simulink model "pvwindupfc11"  (R2016a)
settings: Solver=VariableStepAuto  StartTime=0.0  StopTime=0.5  RelTol=1e-3
undefined symbols (not defined in the file): BCMS11, c1, c2, c3, c4, c5, c6, Clink_3L, DiscIntNeverNeededParam, fdesignblkfcn, Fnom, gcbh, Ion, Ki_Ireg_3L, Ki_VDCreg_3L, Kp_Ireg_3L, Kp_VDCreg_3L, LimitL_Ireg_3L, LimitL_VDCreg_3L, LimitU_Ireg_3L, LimitU_VDCreg_3L, Lithium, LowerLimit, Pnom_3L, Pnom_dc_3L, PV11, Ts_Control, Ts_Power, Ts_PWM, UpperLimit, Vnom_dc_3L, Vnom_prim_3L, Vnom_sec_3L
libraries: powerlib x98, powerlib_extras x29, powerlib_meascontrol x20, fuzblock x2, simulink x1, electricdrivelib x1
(part 3 of 4)

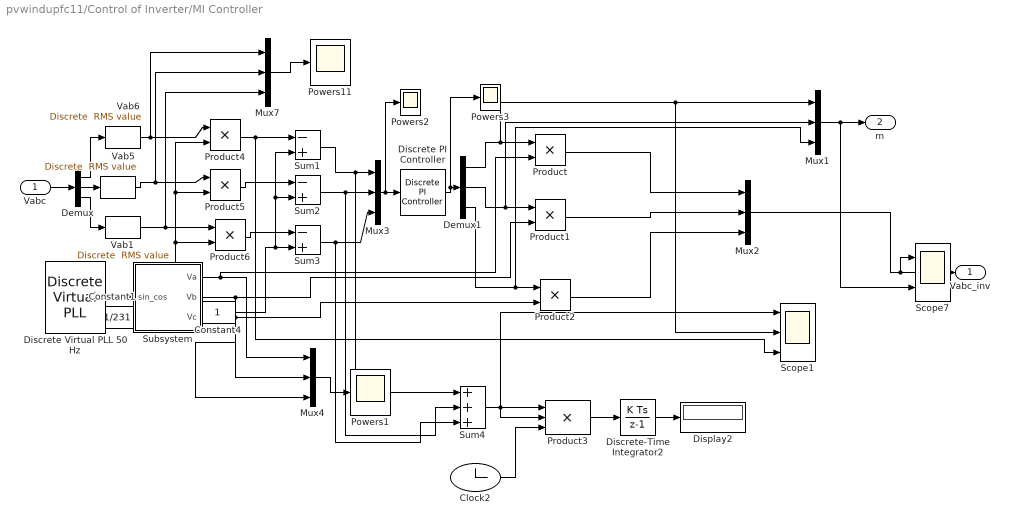
== system pvwindupfc11/Control of Inverter/MI Controller ==
  Vabc : Inport
  Clock2 : Clock
  Constant1 : Constant  Value=1/231
  Constant4 : Constant
  Demux : Demux  Outputs=3
  Demux1 : Demux  Outputs=3
  Discrete PI Controller : powerlib_extras/Discrete  Control Blocks/Discrete PI Controller  Kp=2  Ki=42  Par_Limits=[1.5 -1]  Init=0  Ts=20e-6
  Discrete Virtual PLL 50 Hz : powerlib_extras/Discrete  Control Blocks/Discrete Virtual PLL  Freq=50  Phase=0  Ts=20e-6
  Discrete-Time Integrator2 : DiscreteIntegrator  SampleTime=20e-6  UpperSaturationLimit=UpperLimit  LowerSaturationLimit=LowerLimit  ICPrevOutput=DiscIntNeverNeededParam  ICPrevScaledInput=DiscIntNeverNeededParam
  Display2 : Display
  Mux{1..4,7} (5 alike) : Mux  Inputs=3
  Powers{1..3,11} (4 alike) : Scope
  Product{,1..2,4..6} (6 alike) : Product  RndMeth=Zero
  Product3 : Product  Inputs=3  SaturateOnIntegerOverflow=on  RndMeth=Zero  InputSameDT=on  OutDataTypeStr=Inherit: Same as first input
  Scope1 : Scope  NumInputPorts=3
  Scope7 : Scope  NumInputPorts=2
  Subsystem : Subsystem
  Sum1 : Sum  Inputs=-+  SaturateOnIntegerOverflow=on  InputSameDT=on  OutDataTypeStr=Inherit: Same as first input
  Sum2 : Sum  Inputs=-+  SaturateOnIntegerOverflow=on  InputSameDT=on  OutDataTypeStr=Inherit: Same as first input
  Sum3 : Sum  Inputs=-+  SaturateOnIntegerOverflow=on  InputSameDT=on  OutDataTypeStr=Inherit: Same as first input
  Sum4 : Sum  Inputs=+++  SaturateOnIntegerOverflow=on  InputSameDT=on  OutDataTypeStr=Inherit: Same as first input
  Vab1 : powerlib_extras/Discrete Measurements/Discrete  RMS value  Freq=50  Mag_Init=0  Ts=20e-6
  Vab5 : powerlib_extras/Discrete Measurements/Discrete  RMS value  Freq=50  Mag_Init=0  Ts=20e-6
  Vab6 : powerlib_extras/Discrete Measurements/Discrete  RMS value  Freq=50  Mag_Init=0  Ts=20e-6
  Vabc_inv : Outport
  m : Outport  Port=2
  wires:
  Mux2/1 -> Vabc_inv/1, Scope7/1
  Product/1 -> Mux2/1
  Product1/1 -> Mux2/2
  Product2/1 -> Mux2/3
  Mux1/1 -> m/1, Scope7/2
  Vab5/1 -> Mux7/2, Product5/1
  Vab1/1 -> Mux7/3, Product6/1
  Constant4/1 -> Sum3/2, Sum2/2, Sum1/2
  Sum1/1 -> Mux3/1, Sum4/1
  Vabc/1 -> Demux/1
  Demux/1 -> Vab6/1
  Demux/2 -> Vab5/1
  Demux/3 -> Vab1/1
  Product3/1 -> Discrete-Time Integrator2/1
  Clock2/1 -> Product3/3
  Discrete-Time Integrator2/1 -> Display2/1
  Sum2/1 -> Mux3/2, Sum4/2
  Sum3/1 -> Mux3/3, Sum4/3
  Mux3/1 -> Powers2/1, Discrete PI Controller/1
  Discrete PI Controller/1 -> Powers3/1, Demux1/1
  Demux1/1 -> Product/1, Mux1/1, Scope1/2
  Demux1/2 -> Product1/1, Mux1/2
  Demux1/3 -> Product2/1, Mux1/3
  Product4/1 -> Sum1/1, Scope1/3
  Product5/1 -> Sum2/1
  Product6/1 -> Sum3/1
  Vab6/1 -> Mux7/1, Product4/1
  Mux7/1 -> Powers11/1
  Discrete Virtual PLL 50 Hz/2 -> Subsystem/1(sin_cos)
  Subsystem/1(Va) -> Product/2, Mux4/1
  Subsystem/2(Vb) -> Product1/2, Mux4/2
  Subsystem/3(Vc) -> Product2/2, Mux4/3
  Mux4/1 -> Powers1/1
  Constant1/1 -> Product6/2, Product5/2, Product4/2
  Sum4/1 -> Product3/1, Product3/2, Scope1/1

== system pvwindupfc11/Control of Inverter/Subsystem1 ==
  Ground4 : powerlib/Elements/Ground  LConnTagsString=a
  Mux1 : Mux  Inputs=3
  Mux2 : Mux  Inputs=3
  Mux7 : Mux  Inputs=3
  Vab : powerlib/Measurements/Voltage Measurement  Tag=PoWeRsYsTeMmEaSuReMeNt  PhasorSimulation=off  OutputType=Magnitude  PSBequivalent=0
  Vab1 : powerlib_extras/Discrete Measurements/Discrete  RMS value  Freq=50  Mag_Init=0  Ts=20e-6
  Vab2 : powerlib_extras/Discrete Measurements/Discrete  RMS value  Freq=50  Mag_Init=0  Ts=20e-6
  Vab5 : powerlib_extras/Discrete Measurements/Discrete  RMS value  Freq=50  Mag_Init=0  Ts=20e-6
  Vbc : powerlib/Measurements/Voltage Measurement  Tag=PoWeRsYsTeMmEaSuReMeNt  PhasorSimulation=off  OutputType=Magnitude  PSBequivalent=0
  Vca : powerlib/Measurements/Voltage Measurement  Tag=PoWeRsYsTeMmEaSuReMeNt  PhasorSimulation=off  OutputType=Magnitude  PSBequivalent=0
  a : powerlib/Measurements/Voltage Measurement  Tag=PoWeRsYsTeMmEaSuReMeNt  PhasorSimulation=off  OutputType=Magnitude  PSBequivalent=0
  b : powerlib/Measurements/Voltage Measurement  Tag=PoWeRsYsTeMmEaSuReMeNt  PhasorSimulation=off  OutputType=Magnitude  PSBequivalent=0
  c : powerlib/Measurements/Voltage Measurement  Tag=PoWeRsYsTeMmEaSuReMeNt  PhasorSimulation=off  OutputType=Magnitude  PSBequivalent=0
  A : PMIOPort  Port=1  Side=Left
  B : PMIOPort  Port=2  Side=Left
  C : PMIOPort  Port=3  Side=Left
  Vph : Outport
  VL-L : Outport  Port=2
  Vph_rms : Outport  Port=3
  wires:
  a/1 -> Mux7/1, Vab5/1
  b/1 -> Mux7/2, Vab1/1
  c/1 -> Mux7/3, Vab2/1
  Mux7/1 -> Vph/1
  Vab/1 -> Mux1/1
  Vbc/1 -> Mux1/2
  Vca/1 -> Mux1/3
  Mux1/1 -> VL-L/1
  Vab5/1 -> Mux2/1
  Vab1/1 -> Mux2/2
  Vab2/1 -> Mux2/3
  Mux2/1 -> Vph_rms/1
  connections:
  Ground4/LConn1 -- c/LConn2 -- b/LConn2 -- a/LConn2
  A/RConn1 -- a/LConn1 -- Vab/LConn1 -- Vca/LConn2
  B/RConn1 -- b/LConn1 -- Vab/LConn2 -- Vbc/LConn1
  C/RConn1 -- c/LConn1 -- Vbc/LConn2 -- Vca/LConn1

== system pvwindupfc11/UPFC1/DC ==
  Add : Sum
  VM1 : powerlib/Measurements/Voltage Measurement  PhasorSimulation=off  OutputType=Complex  PSBequivalent=0
  VM2 : powerlib/Measurements/Voltage Measurement  PhasorSimulation=off  OutputType=Complex  PSBequivalent=0
  P : PMIOPort  Port=1  Side=Left
  N : PMIOPort  Port=2  Side=Left
  M : PMIOPort  Port=3  Side=Left
  p : PMIOPort  Port=4  Side=Right
  n : PMIOPort  Port=5  Side=Right
  m : PMIOPort  Port=6  Side=Right
  tag scope: VdcM_3L=global, VdcP_3L=global, Vdc_3L=global
  wires:
  Add/1 -> [Vdc_3L]
  VM2/1 -> [VdcM_3L], Add/2
  VM1/1 -> Add/1, [VdcP_3L]
  connections:
  N/RConn1 -- VM2/LConn1 -- n/RConn1 -- VM1/LConn2
  M/RConn1 -- m/RConn1 -- VM2/LConn2
  P/RConn1 -- p/RConn1 -- VM1/LConn1

== system pvwindupfc11/UPFC1/DC_ ==
  Add : Sum
  VM1 : powerlib/Measurements/Voltage Measurement  PhasorSimulation=off  OutputType=Complex  PSBequivalent=0
  VM2 : powerlib/Measurements/Voltage Measurement  PhasorSimulation=off  OutputType=Complex  PSBequivalent=0
  P : PMIOPort  Port=1  Side=Left
  N : PMIOPort  Port=2  Side=Left
  M : PMIOPort  Port=3  Side=Left
  p : PMIOPort  Port=4  Side=Right
  n : PMIOPort  Port=5  Side=Right
  m : PMIOPort  Port=6  Side=Right
  tag scope: VdcM_inv=global, VdcP_inv=global, Vdc_inv=global
  wires:
  Add/1 -> [Vdc_inv]
  VM2/1 -> [VdcM_inv], Add/2
  VM1/1 -> Add/1, [VdcP_inv]
  connections:
  N/RConn1 -- VM2/LConn1 -- n/RConn1 -- VM1/LConn2
  M/RConn1 -- m/RConn1 -- VM2/LConn2
  P/RConn1 -- p/RConn1 -- VM1/LConn1

== system pvwindupfc11/UPFC1/Imes_SH ==
  Current Measurement : powerlib/Measurements/Current Measurement  Tag=PoWeRsYsTeMmEaSuReMeNt  PhasorSimulation=off  OutputType=Magnitude  PSBequivalent=0
  Current Measurement1 : powerlib/Measurements/Current Measurement  Tag=PoWeRsYsTeMmEaSuReMeNt  PhasorSimulation=off  OutputType=Magnitude  PSBequivalent=0
  Current Measurement2 : powerlib/Measurements/Current Measurement  Tag=PoWeRsYsTeMmEaSuReMeNt  PhasorSimulation=off  OutputType=Magnitude  PSBequivalent=0
  Mux : Mux  Inputs=3
  "A " : PMIOPort  Port=1  Side=Left
  "B " : PMIOPort  Port=2  Side=Left
  "C " : PMIOPort  Port=3  Side=Left
  " A" : PMIOPort  Port=4  Side=Right
  " B" : PMIOPort  Port=5  Side=Right
  " C" : PMIOPort  Port=6  Side=Right
  tag scope: Iabc_SH=global
  wires:
  Current Measurement1/1 -> Mux/2
  Current Measurement2/1 -> Mux/3
  Current Measurement/1 -> Mux/1
  Mux/1 -> [Iabc_SH]
  connections:
  Current Measurement2/RConn1 -- " C"/RConn1
  "C "/RConn1 -- Current Measurement2/LConn1
  Current Measurement1/RConn1 -- " B"/RConn1
  "B "/RConn1 -- Current Measurement1/LConn1
  Current Measurement/RConn1 -- " A"/RConn1
  "A "/RConn1 -- Current Measurement/LConn1

== system pvwindupfc11/UPFC1/Imes_Se ==
  Current Measurement : powerlib/Measurements/Current Measurement  Tag=PoWeRsYsTeMmEaSuReMeNt  PhasorSimulation=off  OutputType=Magnitude  PSBequivalent=0
  Current Measurement1 : powerlib/Measurements/Current Measurement  Tag=PoWeRsYsTeMmEaSuReMeNt  PhasorSimulation=off  OutputType=Magnitude  PSBequivalent=0
  Current Measurement2 : powerlib/Measurements/Current Measurement  Tag=PoWeRsYsTeMmEaSuReMeNt  PhasorSimulation=off  OutputType=Magnitude  PSBequivalent=0
  Mux : Mux  Inputs=3
  "A " : PMIOPort  Port=1  Side=Left
  "B " : PMIOPort  Port=2  Side=Left
  "C " : PMIOPort  Port=3  Side=Left
  " A" : PMIOPort  Port=4  Side=Right
  " B" : PMIOPort  Port=5  Side=Right
  " C" : PMIOPort  Port=6  Side=Right
  tag scope: Iabc_SE=global
  wires:
  Current Measurement1/1 -> Mux/2
  Current Measurement2/1 -> Mux/3
  Current Measurement/1 -> Mux/1
  Mux/1 -> [Iabc_SE]
  connections:
  Current Measurement2/RConn1 -- " C"/RConn1
  "C "/RConn1 -- Current Measurement2/LConn1
  Current Measurement1/RConn1 -- " B"/RConn1
  "B "/RConn1 -- Current Measurement1/LConn1
  Current Measurement/RConn1 -- " A"/RConn1
  "A "/RConn1 -- Current Measurement/LConn1

== system pvwindupfc11/Wind-MPPT/Current Controller1 ==
  Iref : Inport
  Ia : Inport  Port=2
  Relay : Relay  OnSwitchValue=h/2  OffSwitchValue=-h/2
  Sum1 : Sum  Inputs=-+  SaturateOnIntegerOverflow=on  InputSameDT=on  OutDataTypeStr=Inherit: Same as first input
  g : Outport  InitialOutput=0
  error1 : Outport  Port=2  InitialOutput=0
  wires:
  Relay/1 -> g/1
  Ia/1 -> Sum1/1
  Iref/1 -> Sum1/2
  Sum1/1 -> Relay/1, error1/1

== system pvwindupfc11/Wind-MPPT/Subsystem ==
  Tref : Inport
  wm : Inport  Port=2
  Vd : Inport  Port=3
  Avoid division by zero : Saturate  UpperLimit=1e6  LowerLimit=1e-6
  Base Torque1 : Product  Inputs=*/  RndMeth=Zero
  Product1 : Product  RndMeth=Zero
  Id_ref : Outport
  wires:
  Product1/1 -> Base Torque1/1
  Avoid division by zero/1 -> Base Torque1/2
  Tref/1 -> Product1/1
  wm/1 -> Product1/2
  Base Torque1/1 -> Id_ref/1
  Vd/1 -> Avoid division by zero/1

== system pvwindupfc11/Wind-MPPT/Torque reference 1 ==
  wm : Inport
  1\ib1 : Gain  Gain=0.001189  SaturateOnIntegerOverflow=on  OutDataTypeStr=Inherit: Same as input  ParamDataTypeStr=Inherit: Same as input
  1\ib2 : Gain  Gain=0.0197  SaturateOnIntegerOverflow=on  OutDataTypeStr=Inherit: Same as input  ParamDataTypeStr=Inherit: Same as input
  Add : Sum
  Constant2 : Constant  Value=1.791e-3
  Differentiator Filter : Subsystem  DialogController=fdesignblkfcn  InitFcn=fdesignblkfcn(gcbh, {'InitFcn'});  mask(Differentiator Filter){}
      mask help: Design a differentiator filter
      settings: CopyFcn=fdesignblkfcn(gcbh, {'CopyFcn'});
      mask Help: helpview(mapfilelocation('dspblks'), 'dspdifferentiatorfilter')
      mask Display: disp('Differentiator');
  Math Function : Math  Operator=square  SaturateOnIntegerOverflow=on
  Product1 : Product  RndMeth=Zero
  Ref. sat.1 : Saturate  UpperLimit=inf  LowerLimit=0
  Subtract : Sum  Inputs=+-
  Tref : Outport
  wires:
  Math Function/1 -> Product1/1
  Constant2/1 -> Product1/2
  wm/1 -> Math Function/1, Differentiator Filter/1(In), 1\ib1/1
  Ref. sat.1/1 -> Tref/1
  Differentiator Filter/1(Out) -> 1\ib2/1
  1\ib1/1 -> Add/2
  Product1/1 -> Subtract/1
  1\ib2/1 -> Add/1
  Subtract/1 -> Ref. sat.1/1

== system pvwindupfc11/wind/Pitch_angle-controller ==
  wr : Inport
  0-pitch_max : Saturate  UpperLimit=45  LowerLimit=0
  Constant2 : Constant  Value=2
  "Rate Limiter   " : RateLimiter  RisingSlewLimit=2  FallingSlewLimit=-2
  Sum : Sum  Inputs=|+-  SaturateOnIntegerOverflow=on
  genertaor terminal6 : Scope  NumInputPorts=2
  pitch_gain : Gain  Gain=500  SaturateOnIntegerOverflow=on  OutDataTypeStr=Inherit: Same as input  ParamDataTypeStr=Inherit: Same as input
  Pitch_angle : Outport
  wires:
  "Rate Limiter   "/1 -> Pitch_angle/1, genertaor terminal6/1
  pitch_gain/1 -> 0-pitch_max/1
  Sum/1 -> pitch_gain/1
  Constant2/1 -> Sum/2
  0-pitch_max/1 -> "Rate Limiter   "/1, genertaor terminal6/2
  wr/1 -> Sum/1

== system pvwindupfc11/wind/Wind Turbine model ==
  Generator speed (pu) : Inport
  Pitch angle (deg) : Inport  Port=2
  Wind speed (m/s) : Inport  Port=3
  1/cp_nom : Gain  Gain=1/cp_nom  SaturateOnIntegerOverflow=on  OutDataTypeStr=Inherit: Same as input  ParamDataTypeStr=Inherit: Same as input
  1/wind_base : Gain  Gain=1/wind_base  SaturateOnIntegerOverflow=on  OutDataTypeStr=Inherit: Same as input  ParamDataTypeStr=Inherit: Same as input
  Avoid division by zero : Saturate  UpperLimit=1e6  LowerLimit=1e-6
  "Avoid division by zero " : Saturate  UpperLimit=1e6  LowerLimit=1e-6
  Gain : Gain  Gain=-1  SaturateOnIntegerOverflow=on  OutDataTypeStr=Inherit: Same as input  ParamDataTypeStr=Inherit: Same as input
  Product : Product  Inputs=/*  SaturateOnIntegerOverflow=on  OutDataTypeStr=Inherit: Same as first input
  "Product " : Product  SaturateOnIntegerOverflow=on  OutDataTypeStr=Inherit: Same as first input
  Product2 : Product  Inputs=*/  SaturateOnIntegerOverflow=on  InputSameDT=on  OutDataTypeStr=Inherit: Same as first input
  Saturation1 : Saturate  UpperLimit=inf  LowerLimit=1e-6
  Scope : Scope
  cp(lambda,beta) : Subsystem
  lambda_nom : Gain  Gain=lambda_nom  SaturateOnIntegerOverflow=on  OutDataTypeStr=Inherit: Same as input  ParamDataTypeStr=Inherit: Same as input
  pu->pu : Gain  Gain=P_wind_base*Pnom/Pelec_base  SaturateOnIntegerOverflow=on  OutDataTypeStr=Inherit: Same as input  ParamDataTypeStr=Inherit: Same as input
  "pu->pu " : Gain  Gain=1/speed_nom  SaturateOnIntegerOverflow=on  OutDataTypeStr=Inherit: Same as input  ParamDataTypeStr=Inherit: Same as input
  wind_speed^3 : Fcn  Expr=u(1)^3
  Tm (pu) : Outport
  wires:
  Pitch angle (deg)/1 -> cp(lambda,beta)/2(beta)
  pu->pu/1 -> Product2/1
  cp(lambda,beta)/1(cp) -> 1/cp_nom/1
  wind_speed^3/1 -> "Product "/1  "Pwind_pu"
  Product2/1 -> Gain/1
  Avoid division by zero/1 -> Product2/2
  Wind speed (m/s)/1 -> 1/wind_base/1
  Gain/1 -> Tm (pu)/1
  Generator speed (pu)/1 -> Avoid division by zero/1, "pu->pu "/1
  "Product "/1 -> pu->pu/1  "Pm_pu"
  lambda_nom/1 -> Saturation1/1  "lambda"
  1/cp_nom/1 -> "Product "/2  "cp_pu"
  Saturation1/1 -> cp(lambda,beta)/1(lambda), Scope/1
  Product/1 -> lambda_nom/1  "lambda_pu"
  1/wind_base/1 -> wind_speed^3/1, "Avoid division by zero "/1  "wind_speed_pu"
  "Avoid division by zero "/1 -> Product/1
  "pu->pu "/1 -> Product/2

== system pvwindupfc11/Control Systems /REC Control/Anti Aliasing Filters ==
  Vabc : Inport  PortDimensions=3
  "Iabc " : Inport  Port=2  PortDimensions=3
  2nd-Order Filter : powerlib_extras/Discrete  Control Blocks/Discrete  2nd-Order Filter  FilterType=Lowpass  Fo=Fc  Zeta=0.707  Ts=Ts  Initialize=off  Vac_Init=[0.8 -25 60]  Vdc_Init=-0.4  PlotResponse=off  param1=[1 120 0.1]
  2nd-Order Filter{1..5} (5 alike) : powerlib_extras/Discrete  Control Blocks/Discrete  2nd-Order Filter  FilterType=Lowpass  Fo=Fc  Zeta=0.707  Ts=Ts  Initialize=off  Vac_Init=[0.8 -25 60]  Vdc_Init=-0.4  PlotResponse=off  param1=[1 5000 0.1]
  Demux : Demux  Outputs=3
  Demux1 : Demux  Outputs=3
  Mux : Mux  Inputs=3
  Mux1 : Mux  Inputs=3
  " Vabc" : Outport
  Iabc : Outport  Port=2
  wires:
  "Iabc "/1 -> Demux1/1
  Demux1/2 -> 2nd-Order Filter4/1
  Demux1/3 -> 2nd-Order Filter5/1
  2nd-Order Filter5/1 -> Mux1/3
  2nd-Order Filter4/1 -> Mux1/2
  Mux1/1 -> Iabc/1
  2nd-Order Filter3/1 -> Mux1/1
  Demux1/1 -> 2nd-Order Filter3/1
  Demux/2 -> 2nd-Order Filter1/1
  Demux/3 -> 2nd-Order Filter2/1
  2nd-Order Filter2/1 -> Mux/3
  2nd-Order Filter1/1 -> Mux/2
  Mux/1 -> " Vabc"/1
  2nd-Order Filter/1 -> Mux/1
  Vabc/1 -> Demux/1
  Demux/1 -> 2nd-Order Filter/1

== system pvwindupfc11/Control Systems /REC Control/Current_control ==
  idq : Inport
  idq_ref : Inport  Port=2
  Udq : Inport  Port=3
  Add : Sum  Inputs=-+
  Add1 : Sum  Inputs=-+
  Demux : Demux  Outputs=2
  Demux1 : Demux  Outputs=2
  Demux2 : Demux  Outputs=2
  Mux : Mux  Inputs=2
  Mux1 : Mux  Inputs=2
  Mux2 : Mux  Inputs=2
  PI_d : Subsystem  DialogController=POWERSYS.PowerSysDialog  mask(Discrete PI Controller){Kp=Kp_Ireg_3L, Ki=Ki_Ireg_3L, Par_Limits=[ LimitU_Ireg_3L LimitL_Ireg_3L ], Init=0.5, Ts=Ts_Control}
      mask prompts: Kp "Proportional gain (Kp):"; Ki "Integral gain (Ki):"; Par_Limits "Output limits: [ Upper   Lower ]"; Init "Output initial value:"; Ts "Sample time:"
      mask help: This block implements a discrete PI controller.
      mask init:
      | UpperLimit=Par_Limits(1);
      | LowerLimit=Par_Limits(2);
      mask Display: disp('PI');
  PI_d1 : Subsystem  DialogController=POWERSYS.PowerSysDialog  mask(Discrete PI Controller){Kp=Kp_Ireg_3L, Ki=Ki_Ireg_3L, Par_Limits=[ LimitU_Ireg_3L LimitL_Ireg_3L ], Init=0.12, Ts=Ts_Control}
      mask prompts: Kp "Proportional gain (Kp):"; Ki "Integral gain (Ki):"; Par_Limits "Output limits: [ Upper   Lower ]"; Init "Output initial value:"; Ts "Sample time:"
      mask help: This block implements a discrete PI controller.
      mask init:
      | UpperLimit=Par_Limits(1);
      | LowerLimit=Par_Limits(2);
      mask Display: disp('PI');
  Saturation : Saturate  UpperLimit=LimitU_Ireg_3L  LowerLimit=LimitL_Ireg_3L
  Sum : Sum  Inputs=|-+
  Sum1 : Sum  Inputs=|+-
  Vdc_3L{1..2,4,7} (4 alike) : Scope
  udq_con : Outport
  wires:
  idq/1 -> Demux/1
  Udq/1 -> Demux2/1
  Demux1/1 -> Mux1/2, Sum/2  "id_ref"
  Demux/1 -> Mux1/1, Sum/1  "id"
  Sum/1 -> Vdc_3L7/1, PI_d/1(Error)
  PI_d/1(Out) -> Add/1
  Demux2/1 -> Add/2
  Sum1/1 -> Vdc_3L1/1, PI_d1/1(Error)
  PI_d1/1(Out) -> Add1/1
  Demux2/2 -> Add1/2
  Demux1/2 -> Mux2/2, Sum1/1  "iq_ref"
  Mux/1 -> Saturation/1
  Add/1 -> Mux/1
  Add1/1 -> Mux/2
  Saturation/1 -> udq_con/1
  Demux/2 -> Mux2/1, Sum1/2  "iq"
  idq_ref/1 -> Demux1/1
  Mux2/1 -> Vdc_3L4/1
  Mux1/1 -> Vdc_3L2/1

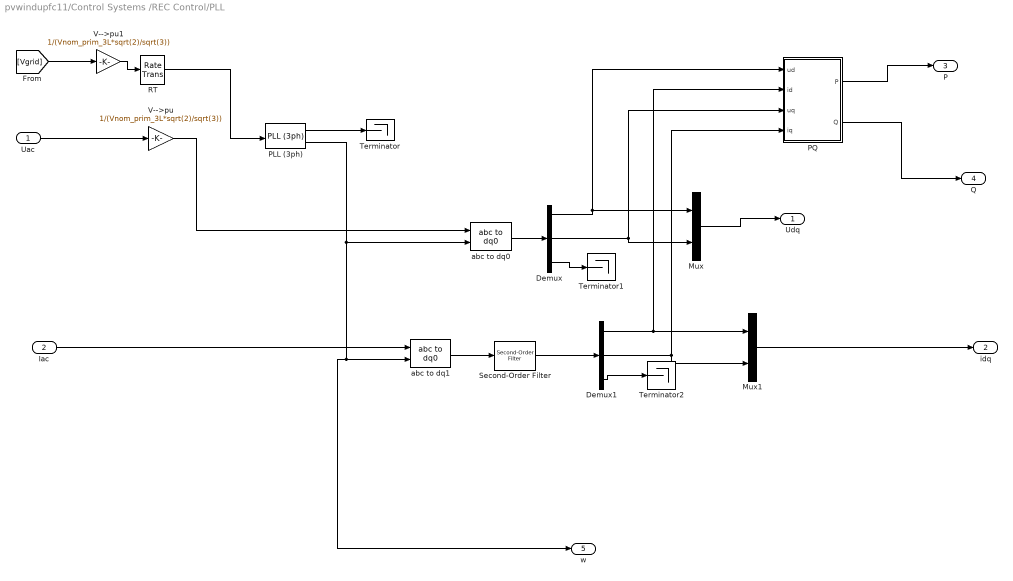
== system pvwindupfc11/Control Systems /REC Control/PLL ==
  Uac : Inport
  Iac : Inport  Port=2
  Demux : Demux  Outputs=3
  Demux1 : Demux  Outputs=3
  Mux : Mux  Inputs=2
  Mux1 : Mux  Inputs=2
  PLL (3ph) : powerlib_meascontrol/PLL/PLL (3ph)  Fmin=45  Par_Init=[0, Fnom]  ParK=[180, 3200, 1]  TcD=1e-4  MaxRateChangeFreq=12  FilterCutOffFreq=25  Ts=Ts_Control  AGC=on
  PQ : Subsystem
  RT : RateTransition  OutPortSampleTime=Ts_Control
  Second-Order Filter : powerlib_meascontrol/Filters/Second-Order Filter  FilterType=Lowpass  Fo=Freq_Filter  Zeta=1  Ts=Ts_Control  Initialize=off  Vac_Init="[0,  0,  60]"  Vdc_Init=0  PlotResponse=off  FreqRange=[0, 500, 1]
  Terminator : Terminator
  Terminator1 : Terminator
  Terminator2 : Terminator
  V-->pu : Gain  Gain=1/(Vnom_prim_3L*sqrt(2)/sqrt(3))
  V-->pu1 : Gain  Gain=1/(Vnom_prim_3L*sqrt(2)/sqrt(3))
  abc to dq0 : powerlib_meascontrol/Transformations/abc to dq0  Alignment=90 degrees behind phase A axis
  abc to dq1 : powerlib_meascontrol/Transformations/abc to dq0  Alignment=90 degrees behind phase A axis
  Udq : Outport
  idq : Outport  Port=2
  P : Outport  Port=3
  Q : Outport  Port=4
  w : Outport  Port=5
  wires:
  Uac/1 -> V-->pu/1
  V-->pu/1 -> abc to dq0/1
  PLL (3ph)/1 -> Terminator/1
  PLL (3ph)/2 -> w/1, abc to dq1/2, abc to dq0/2
  abc to dq0/1 -> Demux/1
  Demux/3 -> Terminator1/1
  Demux/1 -> PQ/1(ud), Mux/1
  Demux/2 -> PQ/3(uq), Mux/2
  Iac/1 -> abc to dq1/1
  abc to dq1/1 -> Second-Order Filter/1
  Demux1/3 -> Terminator2/1
  Demux1/1 -> PQ/2(id), Mux1/1
  Demux1/2 -> Mux1/2, PQ/4(iq)
  Mux/1 -> Udq/1
  Mux1/1 -> idq/1
  PQ/2(Q) -> Q/1
  PQ/1(P) -> P/1
  Second-Order Filter/1 -> Demux1/1
  [Vgrid] -> V-->pu1/1
  V-->pu1/1 -> RT/1
  RT/1 -> PLL (3ph)/1

== system pvwindupfc11/Control Systems /REC Control/PWM Gen 3L ==
  Select : Inport
  Uref : Inport  Port=2
  PWMgen - Averaging : Subsystem
  Pavg_3L : Subsystem
  Switch : Switch  Threshold=1.5
  g : Outport
  wires:
  Select/1 -> PWMgen - Averaging/Enable, Switch/2
  PWMgen - Averaging/1(g1_avg) -> Pavg_3L/1(g1)
  Switch/1 -> g/1
  PWMgen - Averaging/2(g4_avg) -> Pavg_3L/2(g4)
  PWMgen - Averaging/3(P) -> Switch/3
  Uref/1 -> PWMgen - Averaging/1(Uref)
  Pavg_3L/1(g) -> Switch/1

== system pvwindupfc11/Control Systems /REC Control/P_Q ==
  note: 0.25pu/cycle
  note: 0.25pu/cycle
  udq : Inport
  Add : Sum
  Add1 : Sum
  Demux1 : Demux  Outputs=2
  Discrete Mean value1 : powerlib_extras/Discrete Measurements/Discrete  Mean value  Freq=Fnom  Vinit=1  Ts=Ts_Control
  Fcn1 : Fcn  Expr=sqrt(u[1]^2+u[2]^2)  SampleTime=Ts_Control
  Mux3 : Mux  Inputs=2
  Product{2..5} (4 alike) : Product  SaturateOnIntegerOverflow=on  InputSameDT=on  OutDataTypeStr=Inherit: Same as first input
  Product6 : Product  Inputs=*/  SaturateOnIntegerOverflow=on  InputSameDT=on  OutDataTypeStr=Inherit: Same as first input
  "Rate Limiter " : Subsystem  DialogController=POWERSYS.PowerSysDialog  mask(Discrete Rate Limiter){R=10, F=-10, Vinit=-0.55, Ts=Ts_Control}
      mask prompts: R "Rising slew rate:"; F "Falling slew rate:"; Vinit "Initial input:"; Ts "Sample time:"
      mask help: DISCRETE BLOCK : Limit rising and falling rates of signal
      mask init:
      | UpperLimit=R*Ts;
      | LowerLimit=F*Ts;
      | power_initmask();
      mask Help: This block is part of a subset of blocks in the Extras library that does not have documentation associated with it, other than the block mask description.
      mask Display: disp('Discrete\nRate\nLimiter')
  "Rate Limiter  " : Subsystem  DialogController=POWERSYS.PowerSysDialog  mask(Discrete Rate Limiter){R=0.25*50, F=-0.25*50, Vinit=0.3, Ts=Ts_Control}
      mask prompts: R "Rising slew rate:"; F "Falling slew rate:"; Vinit "Initial input:"; Ts "Sample time:"
      mask help: DISCRETE BLOCK : Limit rising and falling rates of signal
      mask init:
      | UpperLimit=R*Ts;
      | LowerLimit=F*Ts;
      | power_initmask();
      mask Help: This block is part of a subset of blocks in the Extras library that does not have documentation associated with it, other than the block mask description.
      mask Display: disp('Discrete\nRate\nLimiter')
  Step : Step  Time=0.9  After=0.3  SampleTime=Ts_Control
  Step1 : Step  Time=1.3  After=-0.3  SampleTime=Ts_Control
  Sum2 : Sum  SaturateOnIntegerOverflow=on  InputSameDT=on  OutDataTypeStr=Inherit: Same as first input
  Sum3 : Sum  Inputs=+-  SaturateOnIntegerOverflow=on  InputSameDT=on  OutDataTypeStr=Inherit: Same as first input
  pref : Constant  Value=-0.55
  qref : Constant  Value=0.3
  idq_ref : Outport
  wires:
  Demux1/1 -> Product5/2, Product2/1
  Demux1/2 -> Product4/2, Product3/1
  Product4/1 -> Sum3/1
  Product2/1 -> Sum2/1
  Product3/1 -> Sum2/2
  Sum3/1 -> Mux3/2
  Product5/1 -> Sum3/2
  Discrete Mean value1/1 -> Product6/2
  Mux3/1 -> Product6/1
  Sum2/1 -> Mux3/1
  "Rate Limiter "/1(Out) -> Product4/1, Product2/2
  "Rate Limiter  "/1(Out) -> Product5/1, Product3/2
  Product6/1 -> idq_ref/1
  udq/1 -> Demux1/1, Fcn1/1
  Fcn1/1 -> Discrete Mean value1/1
  Step/1 -> Add/2
  qref/1 -> Add/1
  Add/1 -> "Rate Limiter  "/1(In)
  pref/1 -> Add1/1
  Add1/1 -> "Rate Limiter "/1(In)
  Step1/1 -> Add1/2

== system pvwindupfc11/Control Systems /REC Control/Scaling ==
  Vdc : Inport
  VdVq : Inport  Port=2
  0.8 to 1.2 x Vnom_dc : Saturate  UpperLimit=1.5*Vnom_dc_3L  LowerLimit=0.5*Vnom_dc_3L
  Constant1 : Constant  Value=Vnom_sec_3L
  Gain1 : Gain  Gain=0.5/sqrt(2)*sqrt(3)
  Product : Product  Inputs=*/
  Product1 : Product  Inputs=**
  VdVq* : Outport
  wires:
  Product1/1 -> VdVq*/1
  VdVq/1 -> Product1/1
  Vdc/1 -> 0.8 to 1.2 x Vnom_dc/1
  Product/1 -> Product1/2
  0.8 to 1.2 x Vnom_dc/1 -> Gain1/1
  Gain1/1 -> Product/2
  Constant1/1 -> Product/1

== system pvwindupfc11/Control Systems /REC Control/Udc_Uac ==
  Udc : Inport
  udq : Inport  Port=2
  Discrete Mean value : powerlib_extras/Discrete Measurements/Discrete  Mean value  Freq=60  Vinit=1  Ts=Ts_Control
  Fcn : Fcn  Expr=sqrt(u[1]^2+u[2]^2)  SampleTime=Ts_Control
  Gain : Gain
  Gain2 : Gain
  Mux : Mux  Inputs=2
  Mux1 : Mux  Inputs=2
  PI_d : Subsystem  DialogController=POWERSYS.PowerSysDialog  mask(Discrete PI Controller){Kp=3, Ki=200, Par_Limits=[1.15 -1.15], Init=0, Ts=Ts_Control}
      mask prompts: Kp "Proportional gain (Kp):"; Ki "Integral gain (Ki):"; Par_Limits "Output limits: [ Upper   Lower ]"; Init "Output initial value:"; Ts "Sample time:"
      mask help: This block implements a discrete PI controller.
      mask init:
      | UpperLimit=Par_Limits(1);
      | LowerLimit=Par_Limits(2);
      mask Display: disp('PI');
  PI_d2 : Subsystem  DialogController=POWERSYS.PowerSysDialog  mask(Discrete PI Controller){Kp=0.5, Ki=50, Par_Limits=[0.1 -0.1], Init=0, Ts=Ts_Control}
      mask prompts: Kp "Proportional gain (Kp):"; Ki "Integral gain (Ki):"; Par_Limits "Output limits: [ Upper   Lower ]"; Init "Output initial value:"; Ts "Sample time:"
      mask help: This block implements a discrete PI controller.
      mask init:
      | UpperLimit=Par_Limits(1);
      | LowerLimit=Par_Limits(2);
      mask Display: disp('PI');
  Saturation1 : Saturate  UpperLimit=1.15  LowerLimit=-1.15
  Sum : Sum  Inputs=|-+
  Sum1 : Sum  Inputs=|++
  Sum4 : Sum  Inputs=|-+
  Udc_ref : Constant
  Udc_ref1 : Constant  Value=0
  Vdc_3L{1..2,4,9} (4 alike) : Scope
  constant : Constant  SampleTime=Ts_Control
  idq_ref : Outport
  wires:
  Sum/1 -> Vdc_3L4/1, PI_d/1(Error)
  Mux/1 -> idq_ref/1
  Udc/1 -> Gain2/1
  Saturation1/1 -> Mux/2
  constant/1 -> Sum4/2
  Sum4/1 -> Vdc_3L9/1, PI_d2/1(Error)
  PI_d2/1(Out) -> Vdc_3L2/1, Gain/1
  Fcn/1 -> Discrete Mean value/1
  udq/1 -> Fcn/1
  Discrete Mean value/1 -> Sum4/1
  Gain/1 -> Sum1/1
  Sum1/1 -> Saturation1/1
  Udc_ref/1 -> Mux1/2, Sum/2
  Gain2/1 -> Mux1/1, Sum/1
  Mux1/1 -> Vdc_3L1/1
  PI_d/1(Out) -> Mux/1

== system pvwindupfc11/Control Systems /SEC Control/PWM Gen 3L ==
  Select : Inport
  Uref : Inport  Port=2
  PWMgen - Averaging : Subsystem
  Pavg_3L : Subsystem
  Switch : Switch  Threshold=1.5
  g : Outport
  wires:
  Select/1 -> PWMgen - Averaging/Enable, Switch/2
  PWMgen - Averaging/1(g1_avg) -> Pavg_3L/1(g1)
  Switch/1 -> g/1
  PWMgen - Averaging/2(g4_avg) -> Pavg_3L/2(g4)
  PWMgen - Averaging/3(P) -> Switch/3
  Uref/1 -> PWMgen - Averaging/1(Uref)
  Pavg_3L/1(g) -> Switch/1

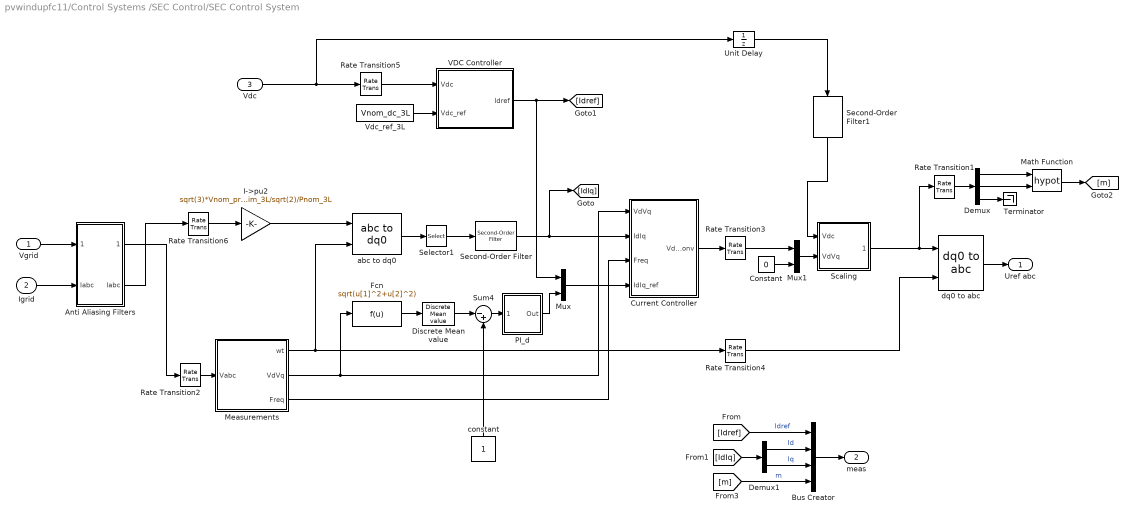
== system pvwindupfc11/Control Systems /SEC Control/SEC Control System ==
  Vgrid : Inport  PortDimensions=3
  Igrid : Inport  Port=2  PortDimensions=3
  Vdc : Inport  Port=3
  Anti Aliasing Filters : Subsystem  mask(Anti-aliasing (2nd order lowpass)){Fc=800, Ts=Ts_Power}
      mask prompts: Fc "Cut-off frequency (Hz):"; Ts "Sample time:"
  Bus Creator : BusCreator  Inputs=4
  Constant : Constant  Value=0
  Current Controller : Subsystem
  Demux : Demux  Outputs=3
  Demux1 : Demux  Outputs=2
  Discrete Mean value : powerlib_extras/Discrete Measurements/Discrete  Mean value  Freq=Fnom  Vinit=1  Ts=Ts_Control
  Fcn : Fcn  Expr=sqrt(u[1]^2+u[2]^2)  SampleTime=Ts_Control
  I->pu2 : Gain  Gain=sqrt(3)*Vnom_prim_3L/sqrt(2)/Pnom_3L  SaturateOnIntegerOverflow=on  OutDataTypeStr=Inherit: Same as input  ParamDataTypeStr=Inherit: Same as input
  Math Function : Math  Operator=hypot  SaturateOnIntegerOverflow=on
  Measurements : Subsystem
  Mux : Mux  Inputs=2
  Mux1 : Mux  Inputs=[2 1]
  PI_d : Subsystem  DialogController=POWERSYS.PowerSysDialog  mask(Discrete PI Controller){Kp=0.5, Ki=50, Par_Limits=[1  -1], Init=0, Ts=Ts_Control}
      mask prompts: Kp "Proportional gain (Kp):"; Ki "Integral gain (Ki):"; Par_Limits "Output limits: [ Upper   Lower ]"; Init "Output initial value:"; Ts "Sample time:"
      mask help: This block implements a discrete PI controller.
      mask init:
      | UpperLimit=Par_Limits(1);
      | LowerLimit=Par_Limits(2);
      mask Display: disp('PI');
  Rate Transition{1..2,5..6} (4 alike) : RateTransition  OutPortSampleTime=Ts_Control
  Rate Transition3 : RateTransition  OutPortSampleTime=Ts_PWM
  Rate Transition4 : RateTransition  OutPortSampleTime=Ts_PWM
  Scaling : Subsystem
  Second-Order Filter : powerlib_meascontrol/Filters/Second-Order Filter  FilterType=Lowpass  Fo=Freq_Filter  Zeta=1  Ts=Ts_Control  Initialize=off  Vac_Init="[0,  0,  60]"  Vdc_Init=0  PlotResponse=off  FreqRange=[0, 500, 1]
  Second-Order Filter1 : powerlib_meascontrol/Filters/Second-Order Filter  FilterType=Lowpass  Fo=Freq_Filter  Zeta=1  Ts=Ts_PWM  Initialize=off  Vac_Init="[0,  0,  60]"  Vdc_Init=0  PlotResponse=off  FreqRange=[0, 500, 1]
  Selector1 : Selector  InputPortWidth=3  IndexOptions=Index vector (dialog)  Indices=[1 2]  OutputSizes=1
  Sum4 : Sum  Inputs=|-+
  Terminator : Terminator
  Unit Delay : UnitDelay  SampleTime=Ts_PWM
  VDC Controller : Subsystem
  Vdc_ref_3L : Constant  Value=Vnom_dc_3L
  abc to dq0 : powerlib_meascontrol/Transformations/abc to dq0  Alignment=90 degrees behind phase A axis
  constant : Constant  SampleTime=Ts_Control
  dq0 to abc : powerlib_meascontrol/Transformations/dq0 to abc  Alignment=90 degrees behind phase A axis
  Uref abc : Outport
  meas : Outport  Port=2
  wires:
  Selector1/1 -> Second-Order Filter/1
  I->pu2/1 -> abc to dq0/1
  abc to dq0/1 -> Selector1/1
  VDC Controller/1(Idref) -> [Idref], Mux/1
  Scaling/1(VdVq*) -> dq0 to abc/1, Rate Transition1/1
  Mux1/1 -> Scaling/2(VdVq)
  Mux/1 -> Current Controller/4(IdIq_ref)
  Demux/3 -> Terminator/1
  Demux/2 -> Math Function/2
  Demux/1 -> Math Function/1
  Constant/1 -> Mux1/2
  Rate Transition3/1 -> Mux1/1
  Rate Transition4/1 -> dq0 to abc/2
  Current Controller/1(VdVq_conv) -> Rate Transition3/1
  dq0 to abc/1 -> Uref abc/1
  Rate Transition2/1 -> Measurements/1(Vabc)
  Rate Transition6/1 -> I->pu2/1
  Measurements/1(wt) -> Rate Transition4/1, abc to dq0/2
  Measurements/2(VdVq) -> Current Controller/1(VdVq), Fcn/1
  Measurements/3(Freq) -> Current Controller/3(Freq)
  Vdc_ref_3L/1 -> VDC Controller/2(Vdc_ref)
  [Idref] -> Bus Creator/1  "Idref"
  Demux1/1 -> Bus Creator/2  "Id"
  Demux1/2 -> Bus Creator/3  "Iq"
  [m] -> Bus Creator/4  "m"
  [IdIq] -> Demux1/1
  Bus Creator/1 -> meas/1
  Math Function/1 -> [m]
  Rate Transition5/1 -> VDC Controller/1(Vdc)
  Rate Transition1/1 -> Demux/1
  Vdc/1 -> Unit Delay/1, Rate Transition5/1
  Unit Delay/1 -> Second-Order Filter1/1
  Second-Order Filter/1 -> [IdIq], Current Controller/2(IdIq)
  Second-Order Filter1/1 -> Scaling/1(Vdc)
  Fcn/1 -> Discrete Mean value/1
  Discrete Mean value/1 -> Sum4/1
  constant/1 -> Sum4/2
  Sum4/1 -> PI_d/1(Error)
  PI_d/1(Out) -> Mux/2
  Vgrid/1 -> Anti Aliasing Filters/1(Vabc)
  Igrid/1 -> Anti Aliasing Filters/2("Iabc ")
  Anti Aliasing Filters/1(" Vabc") -> Rate Transition2/1
  Anti Aliasing Filters/2(Iabc) -> Rate Transition6/1

== system pvwindupfc11/Control of Inverter/MI Controller/Subsystem ==
  sin_cos : Inport  PortDimensions=2
  Demux : Demux  Outputs=2
  Fcn2 : Fcn  Expr=1*u[1]
  Fcn4 : Fcn  Expr=1*u[3]
  Fcn5 : Fcn  Expr=1*u[5]
  K1 : Constant  Value=0.5
  K2 : Constant  Value=sqrt(3)/2
  Mux2 : Mux  Inputs=6
  Product{,1..3} (4 alike) : Product  SaturateOnIntegerOverflow=on  InputSameDT=on  OutDataTypeStr=Inherit: Same as first input
  Sum : Sum  Inputs=--  SaturateOnIntegerOverflow=on  InputSameDT=on  OutDataTypeStr=Inherit: Same as first input
  Sum1 : Sum  Inputs=-+  SaturateOnIntegerOverflow=on  InputSameDT=on  OutDataTypeStr=Inherit: Same as first input
  Sum2 : Sum  Inputs=--  SaturateOnIntegerOverflow=on  InputSameDT=on  OutDataTypeStr=Inherit: Same as first input
  Sum3 : Sum  Inputs=--  SaturateOnIntegerOverflow=on  InputSameDT=on  OutDataTypeStr=Inherit: Same as first input
  Va : Outport
  Vb : Outport  Port=2
  Vc : Outport  Port=3
  wires:
  sin_cos/1 -> Demux/1
  Demux/1 -> Product/1, Product2/1, Sum2/2, Mux2/1  "sin(wt)"
  Product/1 -> Sum/1
  Product1/1 -> Sum/2
  Product3/1 -> Sum1/1
  Product2/1 -> Sum1/2
  Sum3/1 -> Mux2/6  "cos(wt+2pi/3)"
  Sum2/1 -> Mux2/5  "sin(wt+2pi/3)"
  K1/1 -> Product/2, Product3/2
  K2/1 -> Product1/2, Product2/2
  Sum/1 -> Mux2/3, Sum2/1  "sin(wt-2pi/3)"
  Sum1/1 -> Mux2/4, Sum3/1  "cos(wt-2pi/3)"
  Demux/2 -> Sum3/2, Product3/1, Product1/1, Mux2/2  "cos(wt)"
  Mux2/1 -> Fcn2/1, Fcn4/1, Fcn5/1
  Fcn2/1 -> Va/1
  Fcn4/1 -> Vb/1
  Fcn5/1 -> Vc/1

== system pvwindupfc11/Wind-MPPT/Torque reference 1/Differentiator Filter ==
  In : Inport
  Generated Filter Block : Subsystem  Tag=FilterWizardSubSystem
      settings: ErrorFcn=dspFilterRealizedInBasicElemsAlgLoopErrFcnCallback
  Out : Outport
  wires:
  Generated Filter Block/1(Output) -> Out/1
  In/1 -> Generated Filter Block/1(Input)

== system pvwindupfc11/wind/Wind Turbine model/cp(lambda,beta) ==
  lambda : Inport
  beta : Inport  Port=2
  Fcn : Fcn  Expr=1/(1/(u[1]+0.08*u[2])-0.035/(u[2]^3+1))
  Fcn1 : Fcn  Expr=c1*(c2/u[2]-c3*u[3]-c4)*exp(-c5/u[2])+c6*u[1]
  Mux : Mux  Inputs=2
  Mux1 : Mux  Inputs=3
  cp : Outport
  wires:
  Fcn/1 -> Mux1/2  "lambda_i"
  Fcn1/1 -> cp/1
  lambda/1 -> Mux1/1, Mux/1
  Mux1/1 -> Fcn1/1
  beta/1 -> Mux1/3, Mux/2
  Mux/1 -> Fcn/1

== system pvwindupfc11/Control Systems /REC Control/Current_control/PI_d ==
  Error : Inport  SampleTime=Ts
  Discrete-Time Integrator : DiscreteIntegrator  InitialCondition=Init  SampleTime=Ts  LimitOutput=on  UpperSaturationLimit=UpperLimit  LowerSaturationLimit=LowerLimit  ICPrevOutput=DiscIntNeverNeededParam  ICPrevScaledInput=DiscIntNeverNeededParam
  Kp4 : Gain  Gain=Kp  SampleTime=Ts  SaturateOnIntegerOverflow=on  OutDataTypeStr=Inherit: Same as input  ParamDataTypeStr=Inherit: Same as input
  Kp5 : Gain  Gain=Ki  SampleTime=Ts  SaturateOnIntegerOverflow=on  OutDataTypeStr=Inherit: Same as input  ParamDataTypeStr=Inherit: Same as input
  Saturation2 : Saturate  UpperLimit=UpperLimit  LowerLimit=LowerLimit  SampleTime=Ts
  Sum6 : Sum  SampleTime=Ts  SaturateOnIntegerOverflow=on  InputSameDT=on  OutDataTypeStr=Inherit: Same as first input
  Zero-Order Hold : ZeroOrderHold  SampleTime=Ts
  Out : Outport  SampleTime=Ts  InitialOutput=0
  wires:
  Saturation2/1 -> Out/1
  Error/1 -> Kp4/1, Kp5/1
  Sum6/1 -> Saturation2/1
  Kp5/1 -> Discrete-Time Integrator/1
  Kp4/1 -> Zero-Order Hold/1
  Discrete-Time Integrator/1 -> Sum6/2
  Zero-Order Hold/1 -> Sum6/1

== system pvwindupfc11/Control Systems /REC Control/Current_control/PI_d1 ==
  Error : Inport  SampleTime=Ts
  Discrete-Time Integrator : DiscreteIntegrator  InitialCondition=Init  SampleTime=Ts  LimitOutput=on  UpperSaturationLimit=UpperLimit  LowerSaturationLimit=LowerLimit  ICPrevOutput=DiscIntNeverNeededParam  ICPrevScaledInput=DiscIntNeverNeededParam
  Kp4 : Gain  Gain=Kp  SampleTime=Ts  SaturateOnIntegerOverflow=on  OutDataTypeStr=Inherit: Same as input  ParamDataTypeStr=Inherit: Same as input
  Kp5 : Gain  Gain=Ki  SampleTime=Ts  SaturateOnIntegerOverflow=on  OutDataTypeStr=Inherit: Same as input  ParamDataTypeStr=Inherit: Same as input
  Saturation2 : Saturate  UpperLimit=UpperLimit  LowerLimit=LowerLimit  SampleTime=Ts
  Sum6 : Sum  SampleTime=Ts  SaturateOnIntegerOverflow=on  InputSameDT=on  OutDataTypeStr=Inherit: Same as first input
  Zero-Order Hold : ZeroOrderHold  SampleTime=Ts
  Out : Outport  SampleTime=Ts  InitialOutput=0
  wires:
  Saturation2/1 -> Out/1
  Error/1 -> Kp4/1, Kp5/1
  Sum6/1 -> Saturation2/1
  Kp5/1 -> Discrete-Time Integrator/1
  Kp4/1 -> Zero-Order Hold/1
  Discrete-Time Integrator/1 -> Sum6/2
  Zero-Order Hold/1 -> Sum6/1

== system pvwindupfc11/Control Systems /REC Control/PLL/PQ ==
  ud : Inport
  id : Inport  Port=2
  uq : Inport  Port=3
  iq : Inport  Port=4
  Add : Sum
  Add1 : Sum  Inputs=+-
  Product{,1..3} (4 alike) : Product
  P : Outport
  Q : Outport  Port=2
  wires:
  id/1 -> Product2/2, Product/2
  Product/1 -> Add/1
  iq/1 -> Product3/1, Product1/2
  uq/1 -> Product2/1, Product1/1
  Product1/1 -> Add/2
  Add/1 -> P/1
  ud/1 -> Product3/2, Product/1
  Product2/1 -> Add1/1
  Product3/1 -> Add1/2
  Add1/1 -> Q/1

== system pvwindupfc11/Control Systems /REC Control/PWM Gen 3L/PWMgen - Averaging ==
  Uref : Inport
  Enable : EnablePort
  Mean : powerlib_meascontrol/Measurements/Mean  Freq=1/Ts_Power  Vinit=0  Ts=Ts_PWM
  Mean1 : powerlib_meascontrol/Measurements/Mean  Freq=1/Ts_Power  Vinit=0  Ts=Ts_PWM
  PWM Gen 3L : powerlib_meascontrol/Pulse & Signal Generators/PWM Generator (3-Level)  ModulatorType=Three-phase bridge (12 pulses)  ModulatorMode=Unsynchronized  nF=27  Fc=Fc_3L  ModulatingSignals=off  m=0.8  Freq=60  Phase=0  Ts=Ts_PWM
  Selector2 : Selector  InputPortWidth=12  IndexOptions=Index vector (dialog)  Indices="[1  5  9]"  OutputSizes=1
  Selector3 : Selector  InputPortWidth=12  IndexOptions=Index vector (dialog)  Indices="[1  5  9]+3"  OutputSizes=1
  g1_avg : Outport
  g4_avg : Outport  Port=2
  P : Outport  Port=3
  wires:
  Uref/1 -> PWM Gen 3L/1
  PWM Gen 3L/1 -> P/1, Selector2/1, Selector3/1
  Selector3/1 -> Mean1/1  "g4"
  Selector2/1 -> Mean/1  "g1"
  Mean/1 -> g1_avg/1
  Mean1/1 -> g4_avg/1

== system pvwindupfc11/Control Systems /REC Control/PWM Gen 3L/Pavg_3L ==
  g1 : Inport  SampleTime=Ts_PWM
  g4 : Inport  Port=2  SampleTime=Ts_PWM
  Add1 : Sum  Inputs=-+
  Add2 : Sum  Inputs=-+
  Mux2 : Mux  Inputs=[ 3 3 3 3 ]
  Selector1 : Selector  InputPortWidth=12  IndexOptions=Index vector (dialog)  Indices=[1 4 7 10 2 5 8 11 3 6 9 12]  OutputSizes=1
  Zero-Order Hold1 : ZeroOrderHold  SampleTime=Ts_Power
  Zero-Order Hold2 : ZeroOrderHold  SampleTime=Ts_Power
  k1 : Constant
  k3 : Constant
  g : Outport  SampleTime=Ts_Power
  wires:
  Selector1/1 -> g/1
  Mux2/1 -> Selector1/1
  Add1/1 -> Mux2/2  "2abc"
  Add2/1 -> Mux2/3  "3abc"
  Zero-Order Hold2/1 -> Mux2/4, Add1/1  "4abc"
  k1/1 -> Add1/2
  Zero-Order Hold1/1 -> Mux2/1, Add2/1  "1abc"
  k3/1 -> Add2/2
  g1/1 -> Zero-Order Hold1/1
  g4/1 -> Zero-Order Hold2/1

== system pvwindupfc11/Control Systems /REC Control/P_Q/Rate Limiter  ==
  note: Beat Ronner
      | ABB Industrie AG
      | Turgi, Switzerland
  note: Delta(u)
  In : Inport
  Saturation : Saturate  UpperLimit=UpperLimit  LowerLimit=LowerLimit
  Sum : Sum  Inputs=|++  SaturateOnIntegerOverflow=on  InputSameDT=on  OutDataTypeStr=Inherit: Same as first input
  Sum1 : Sum  Inputs=|+-  SaturateOnIntegerOverflow=on  InputSameDT=on  OutDataTypeStr=Inherit: Same as first input
  Unit Delay : UnitDelay  InitialCondition=Vinit  SampleTime=Ts
  Out : Outport
  wires:
  Unit Delay/1 -> Sum/2, Sum1/2  "y-1"
  Sum/1 -> Unit Delay/1, Out/1  "y"
  Saturation/1 -> Sum/1  "Delta(u)_limit"
  Sum1/1 -> Saturation/1
  In/1 -> Sum1/1  "u"

== system pvwindupfc11/Control Systems /REC Control/P_Q/Rate Limiter   ==
  note: Beat Ronner
      | ABB Industrie AG
      | Turgi, Switzerland
  note: Delta(u)
  In : Inport
  Saturation : Saturate  UpperLimit=UpperLimit  LowerLimit=LowerLimit
  Sum : Sum  Inputs=|++  SaturateOnIntegerOverflow=on  InputSameDT=on  OutDataTypeStr=Inherit: Same as first input
  Sum1 : Sum  Inputs=|+-  SaturateOnIntegerOverflow=on  InputSameDT=on  OutDataTypeStr=Inherit: Same as first input
  Unit Delay : UnitDelay  InitialCondition=Vinit  SampleTime=Ts
  Out : Outport
  wires:
  Unit Delay/1 -> Sum/2, Sum1/2  "y-1"
  Sum/1 -> Unit Delay/1, Out/1  "y"
  Saturation/1 -> Sum/1  "Delta(u)_limit"
  Sum1/1 -> Saturation/1
  In/1 -> Sum1/1  "u"

== system pvwindupfc11/Control Systems /REC Control/Udc_Uac/PI_d ==
  Error : Inport  SampleTime=Ts
  Discrete-Time Integrator : DiscreteIntegrator  InitialCondition=Init  SampleTime=Ts  LimitOutput=on  UpperSaturationLimit=UpperLimit  LowerSaturationLimit=LowerLimit  ICPrevOutput=DiscIntNeverNeededParam  ICPrevScaledInput=DiscIntNeverNeededParam
  Kp4 : Gain  Gain=Kp  SampleTime=Ts  SaturateOnIntegerOverflow=on  OutDataTypeStr=Inherit: Same as input  ParamDataTypeStr=Inherit: Same as input
  Kp5 : Gain  Gain=Ki  SampleTime=Ts  SaturateOnIntegerOverflow=on  OutDataTypeStr=Inherit: Same as input  ParamDataTypeStr=Inherit: Same as input
  Saturation2 : Saturate  UpperLimit=UpperLimit  LowerLimit=LowerLimit  SampleTime=Ts
  Sum6 : Sum  SampleTime=Ts  SaturateOnIntegerOverflow=on  InputSameDT=on  OutDataTypeStr=Inherit: Same as first input
  Zero-Order Hold : ZeroOrderHold  SampleTime=Ts
  Out : Outport  SampleTime=Ts  InitialOutput=0
  wires:
  Saturation2/1 -> Out/1
  Error/1 -> Kp4/1, Kp5/1
  Sum6/1 -> Saturation2/1
  Kp5/1 -> Discrete-Time Integrator/1
  Kp4/1 -> Zero-Order Hold/1
  Discrete-Time Integrator/1 -> Sum6/2
  Zero-Order Hold/1 -> Sum6/1

== system pvwindupfc11/Control Systems /REC Control/Udc_Uac/PI_d2 ==
  Error : Inport  SampleTime=Ts
  Discrete-Time Integrator : DiscreteIntegrator  InitialCondition=Init  SampleTime=Ts  LimitOutput=on  UpperSaturationLimit=UpperLimit  LowerSaturationLimit=LowerLimit  ICPrevOutput=DiscIntNeverNeededParam  ICPrevScaledInput=DiscIntNeverNeededParam
  Kp4 : Gain  Gain=Kp  SampleTime=Ts  SaturateOnIntegerOverflow=on  OutDataTypeStr=Inherit: Same as input  ParamDataTypeStr=Inherit: Same as input
  Kp5 : Gain  Gain=Ki  SampleTime=Ts  SaturateOnIntegerOverflow=on  OutDataTypeStr=Inherit: Same as input  ParamDataTypeStr=Inherit: Same as input
  Saturation2 : Saturate  UpperLimit=UpperLimit  LowerLimit=LowerLimit  SampleTime=Ts
  Sum6 : Sum  SampleTime=Ts  SaturateOnIntegerOverflow=on  InputSameDT=on  OutDataTypeStr=Inherit: Same as first input
  Zero-Order Hold : ZeroOrderHold  SampleTime=Ts
  Out : Outport  SampleTime=Ts  InitialOutput=0
  wires:
  Saturation2/1 -> Out/1
  Error/1 -> Kp4/1, Kp5/1
  Sum6/1 -> Saturation2/1
  Kp5/1 -> Discrete-Time Integrator/1
  Kp4/1 -> Zero-Order Hold/1
  Discrete-Time Integrator/1 -> Sum6/2
  Zero-Order Hold/1 -> Sum6/1

== system pvwindupfc11/Control Systems /SEC Control/PWM Gen 3L/PWMgen - Averaging ==
  Uref : Inport
  Enable : EnablePort
  Mean : powerlib_meascontrol/Measurements/Mean  Freq=1/Ts_Power  Vinit=0  Ts=Ts_PWM
  Mean1 : powerlib_meascontrol/Measurements/Mean  Freq=1/Ts_Power  Vinit=0  Ts=Ts_PWM
  PWM Gen 3L : powerlib_meascontrol/Pulse & Signal Generators/PWM Generator (3-Level)  ModulatorType=Three-phase bridge (12 pulses)  ModulatorMode=Unsynchronized  nF=27  Fc=Fc_3L  ModulatingSignals=off  m=0.8  Freq=60  Phase=0  Ts=Ts_PWM
  Selector2 : Selector  InputPortWidth=12  IndexOptions=Index vector (dialog)  Indices="[1  5  9]"  OutputSizes=1
  Selector3 : Selector  InputPortWidth=12  IndexOptions=Index vector (dialog)  Indices="[1  5  9]+3"  OutputSizes=1
  g1_avg : Outport
  g4_avg : Outport  Port=2
  P : Outport  Port=3
  wires:
  Uref/1 -> PWM Gen 3L/1
  PWM Gen 3L/1 -> P/1, Selector2/1, Selector3/1
  Selector3/1 -> Mean1/1  "g4"
  Selector2/1 -> Mean/1  "g1"
  Mean/1 -> g1_avg/1
  Mean1/1 -> g4_avg/1

== system pvwindupfc11/Control Systems /SEC Control/PWM Gen 3L/Pavg_3L ==
  g1 : Inport  SampleTime=Ts_PWM
  g4 : Inport  Port=2  SampleTime=Ts_PWM
  Add1 : Sum  Inputs=-+
  Add2 : Sum  Inputs=-+
  Mux2 : Mux  Inputs=[ 3 3 3 3 ]
  Selector1 : Selector  InputPortWidth=12  IndexOptions=Index vector (dialog)  Indices=[1 4 7 10 2 5 8 11 3 6 9 12]  OutputSizes=1
  Zero-Order Hold1 : ZeroOrderHold  SampleTime=Ts_Power
  Zero-Order Hold2 : ZeroOrderHold  SampleTime=Ts_Power
  k1 : Constant
  k3 : Constant
  g : Outport  SampleTime=Ts_Power
  wires:
  Selector1/1 -> g/1
  Mux2/1 -> Selector1/1
  Add1/1 -> Mux2/2  "2abc"
  Add2/1 -> Mux2/3  "3abc"
  Zero-Order Hold2/1 -> Mux2/4, Add1/1  "4abc"
  k1/1 -> Add1/2
  Zero-Order Hold1/1 -> Mux2/1, Add2/1  "1abc"
  k3/1 -> Add2/2
  g1/1 -> Zero-Order Hold1/1
  g4/1 -> Zero-Order Hold2/1

== system pvwindupfc11/Control Systems /SEC Control/SEC Control System/Anti Aliasing Filters ==
  Vabc : Inport  PortDimensions=3
  "Iabc " : Inport  Port=2  PortDimensions=3
  2nd-Order Filter : powerlib_extras/Discrete  Control Blocks/Discrete  2nd-Order Filter  FilterType=Lowpass  Fo=Fc  Zeta=0.707  Ts=Ts  Initialize=off  Vac_Init=[0.8 -25 60]  Vdc_Init=-0.4  PlotResponse=off  param1=[1 120 0.1]
  2nd-Order Filter{1..5} (5 alike) : powerlib_extras/Discrete  Control Blocks/Discrete  2nd-Order Filter  FilterType=Lowpass  Fo=Fc  Zeta=0.707  Ts=Ts  Initialize=off  Vac_Init=[0.8 -25 60]  Vdc_Init=-0.4  PlotResponse=off  param1=[1 5000 0.1]
  Demux : Demux  Outputs=3
  Demux1 : Demux  Outputs=3
  Mux : Mux  Inputs=3
  Mux1 : Mux  Inputs=3
  " Vabc" : Outport
  Iabc : Outport  Port=2
  wires:
  "Iabc "/1 -> Demux1/1
  Demux1/2 -> 2nd-Order Filter4/1
  Demux1/3 -> 2nd-Order Filter5/1
  2nd-Order Filter5/1 -> Mux1/3
  2nd-Order Filter4/1 -> Mux1/2
  Mux1/1 -> Iabc/1
  2nd-Order Filter3/1 -> Mux1/1
  Demux1/1 -> 2nd-Order Filter3/1
  Demux/2 -> 2nd-Order Filter1/1
  Demux/3 -> 2nd-Order Filter2/1
  2nd-Order Filter2/1 -> Mux/3
  2nd-Order Filter1/1 -> Mux/2
  Mux/1 -> " Vabc"/1
  2nd-Order Filter/1 -> Mux/1
  Vabc/1 -> Demux/1
  Demux/1 -> 2nd-Order Filter/1

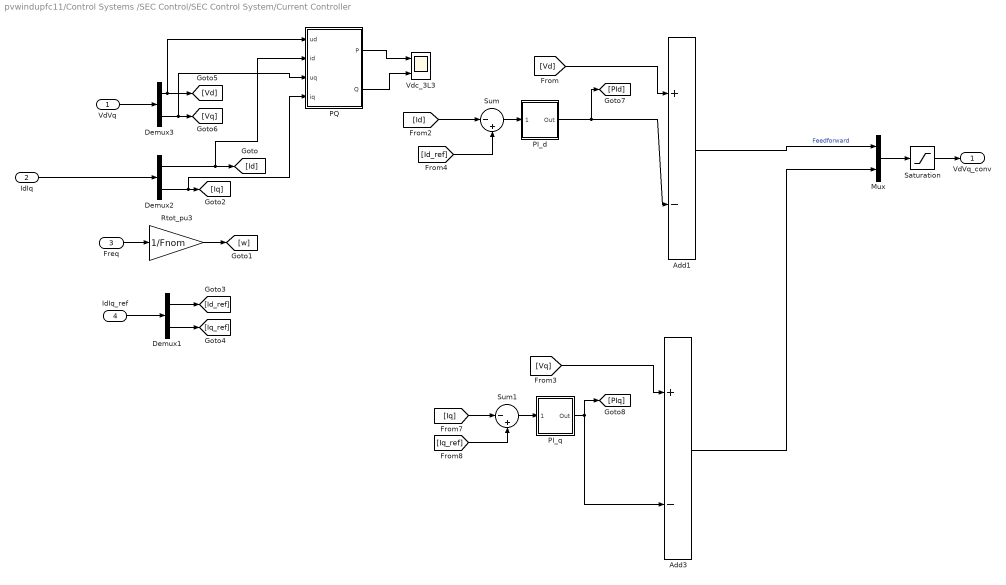
== system pvwindupfc11/Control Systems /SEC Control/SEC Control System/Current Controller ==
  VdVq : Inport  PortDimensions=2
  IdIq : Inport  Port=2  PortDimensions=2
  Freq : Inport  Port=3  PortDimensions=1
  IdIq_ref : Inport  Port=4  PortDimensions=2
  Add1 : Sum  Inputs=+-
  Add3 : Sum  Inputs=+-
  Demux1 : Demux  Outputs=2
  Demux2 : Demux  Outputs=2
  Demux3 : Demux  Outputs=2
  Mux : Mux  Inputs=2
  PI_d : Subsystem  DialogController=POWERSYS.PowerSysDialog  mask(Discrete PI Controller){Kp=Kp_Ireg_3L, Ki=Ki_Ireg_3L, Par_Limits=[ LimitU_Ireg_3L LimitL_Ireg_3L ], Init=0, Ts=Ts_Control}
      mask prompts: Kp "Proportional gain (Kp):"; Ki "Integral gain (Ki):"; Par_Limits "Output limits: [ Upper   Lower ]"; Init "Output initial value:"; Ts "Sample time:"
      mask help: This block implements a discrete PI controller.
      mask init:
      | UpperLimit=Par_Limits(1);
      | LowerLimit=Par_Limits(2);
      mask Display: disp('PI');
  PI_q : Subsystem  DialogController=POWERSYS.PowerSysDialog  mask(Discrete PI Controller){Kp=Kp_Ireg_3L, Ki=Ki_Ireg_3L, Par_Limits=[ LimitU_Ireg_3L LimitL_Ireg_3L ], Init=0, Ts=Ts_Control}
      mask prompts: Kp "Proportional gain (Kp):"; Ki "Integral gain (Ki):"; Par_Limits "Output limits: [ Upper   Lower ]"; Init "Output initial value:"; Ts "Sample time:"
      mask help: This block implements a discrete PI controller.
      mask init:
      | UpperLimit=Par_Limits(1);
      | LowerLimit=Par_Limits(2);
      mask Display: disp('PI');
  PQ : Subsystem
  Rtot_pu3 : Gain  Gain=1/Fnom  SaturateOnIntegerOverflow=on  OutDataTypeStr=Inherit: Same as input  ParamDataTypeStr=Inherit: Same as input
  Saturation : Saturate  UpperLimit=LimitU_Ireg_3L  LowerLimit=LimitL_Ireg_3L
  Sum : Sum  Inputs=|-+
  Sum1 : Sum  Inputs=|-+
  Vdc_3L3 : Scope  NumInputPorts=2
  VdVq_conv : Outport
  wires:
  Add1/1 -> Mux/1  "Feedforward"
  PI_d/1(Out) -> [PId], Add1/2
  PI_q/1(Out) -> [PIq], Add3/2
  [Vd] -> Add1/1
  [Vq] -> Add3/1
  Demux2/1 -> PQ/2(id), [Id]
  IdIq/1 -> Demux2/1
  Saturation/1 -> VdVq_conv/1
  [Id] -> Sum/1
  [Iq] -> Sum1/1
  Demux2/2 -> PQ/4(iq), [Iq]
  Add3/1 -> Mux/2
  [Iq_ref] -> Sum1/2
  Sum1/1 -> PI_q/1(Error)
  [Id_ref] -> Sum/2
  Sum/1 -> PI_d/1(Error)
  Mux/1 -> Saturation/1
  VdVq/1 -> Demux3/1
  Demux3/2 -> PQ/3(uq), [Vq]
  Demux3/1 -> [Vd], PQ/1(ud)
  IdIq_ref/1 -> Demux1/1
  Demux1/2 -> [Iq_ref]
  Demux1/1 -> [Id_ref]
  Rtot_pu3/1 -> [w]
  Freq/1 -> Rtot_pu3/1
  PQ/1(P) -> Vdc_3L3/1
  PQ/2(Q) -> Vdc_3L3/2

== system pvwindupfc11/Control Systems /SEC Control/SEC Control System/Measurements ==
  Vabc : Inport  PortDimensions=3
  PLL (3ph) : powerlib_meascontrol/PLL/PLL (3ph)  Fmin=45  Par_Init=[0, Fnom]  ParK=[180, 3200, 0]/2  TcD=1e-4  MaxRateChangeFreq=12  FilterCutOffFreq=25  Ts=Ts_Control  AGC=on
  Selector2 : Selector  InputPortWidth=3  IndexOptions=Index vector (dialog)  Indices=[1 2]  OutputSizes=1
  V->pu1 : Gain  Gain=1/(Vnom_prim_3L*sqrt(2)/sqrt(3))  SaturateOnIntegerOverflow=on  OutDataTypeStr=Inherit: Same as input  ParamDataTypeStr=Inherit: Same as input
  abc to dq1 : powerlib_meascontrol/Transformations/abc to dq0  Alignment=90 degrees behind phase A axis
  wt : Outport
  VdVq : Outport  Port=2
  Freq : Outport  Port=3
  wires:
  Selector2/1 -> VdVq/1
  abc to dq1/1 -> Selector2/1
  PLL (3ph)/1 -> Freq/1
  V->pu1/1 -> PLL (3ph)/1, abc to dq1/1
  Vabc/1 -> V->pu1/1
  PLL (3ph)/2 -> wt/1, abc to dq1/2

== system pvwindupfc11/Control Systems /SEC Control/SEC Control System/PI_d ==
  Error : Inport  SampleTime=Ts
  Discrete-Time Integrator : DiscreteIntegrator  InitialCondition=Init  SampleTime=Ts  LimitOutput=on  UpperSaturationLimit=UpperLimit  LowerSaturationLimit=LowerLimit  ICPrevOutput=DiscIntNeverNeededParam  ICPrevScaledInput=DiscIntNeverNeededParam
  Kp4 : Gain  Gain=Kp  SampleTime=Ts  SaturateOnIntegerOverflow=on  OutDataTypeStr=Inherit: Same as input  ParamDataTypeStr=Inherit: Same as input
  Kp5 : Gain  Gain=Ki  SampleTime=Ts  SaturateOnIntegerOverflow=on  OutDataTypeStr=Inherit: Same as input  ParamDataTypeStr=Inherit: Same as input
  Saturation2 : Saturate  UpperLimit=UpperLimit  LowerLimit=LowerLimit  SampleTime=Ts
  Sum6 : Sum  SampleTime=Ts  SaturateOnIntegerOverflow=on  InputSameDT=on  OutDataTypeStr=Inherit: Same as first input
  Zero-Order Hold : ZeroOrderHold  SampleTime=Ts
  Out : Outport  SampleTime=Ts  InitialOutput=0
  wires:
  Saturation2/1 -> Out/1
  Error/1 -> Kp4/1, Kp5/1
  Sum6/1 -> Saturation2/1
  Kp5/1 -> Discrete-Time Integrator/1
  Kp4/1 -> Zero-Order Hold/1
  Discrete-Time Integrator/1 -> Sum6/2
  Zero-Order Hold/1 -> Sum6/1
